simulink model "DataCenterCooling"  (R2026a)
settings: Solver=VariableStepAuto  StopTime=432000  AbsTol=1e-3
PreLoadFcn:
  | load DataCenterCoolingHeatLoad.mat
  | load DataCenterCoolingEnviornment.mat
  | 
  | % Chiller Setpoint
  | T_chiller = 18; % degC
  | 
  | % Pipes
  | server_pipe_D = 0.02; % m
  | server_pipe_L = 12; % m
  | server_pipe_thickness = 0.002; % m
  | server_num_pipes = 800;
  | 
  | % Material properties
  | rho_pipe = 7800; % kg/m^3
  | cp_pipe = 500; % J/(kg*K)
  | 
  | % Total connecting port areas
  | port_area = 0.2; % m^2
  | 
  | % Cooling tower
  | T_reservoir = 23; % degC
  | fan_area = 15; % m^2
  | tower_height = 3; % m
  | tower_area = 15; % m^2
libraries: fl_lib x38, nesl_utility x24, SimscapeFluids_lib x14, simulink_extras x2, slpidlib x2
(part 2 of 2)

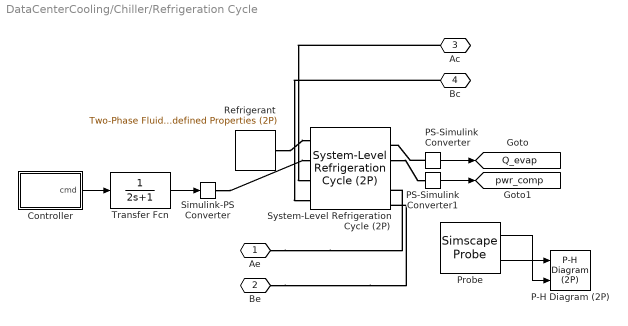
== system DataCenterCooling/Chiller/Refrigeration Cycle ==
  Controller : Subsystem
  P-H Diagram (2P) : SimscapeFluids_lib/Two-Phase Fluid/Utilities/P-H Diagram (2P)  p_unit=MPa  h_unit=kJ/kg
  PS-Simulink Converter : nesl_utility/PS-Simulink Converter  PhysicalDomain=network_engine_domain  SubClassName=ps_output  LeftPortType=input  RightPortType=output  PseudoPeriodic=off  Frequencies=[]  VectorFormat=inherit  Unit=kW  AffineConversion=off
  PS-Simulink Converter1 : nesl_utility/PS-Simulink Converter  PhysicalDomain=network_engine_domain  SubClassName=ps_output  LeftPortType=input  RightPortType=output  PseudoPeriodic=off  Frequencies=[]  VectorFormat=inherit  Unit=kW  AffineConversion=off
  Probe : SimscapeProbe  BoundBlock=48  Variables={h_cycle, p_cycle}
  Refrigerant : SimscapeFluids_lib/Two-Phase Fluid/Utilities/Two-Phase Fluid Predefined Properties (2P)  fluid=fluids.two_phase_fluid.utilities.enum.Fluid.R134a  p_atm=0.101325 MPa  properties_range_check=simscape.enum.assert.action.error  q_rev=0.01 Pa
  Simulink-PS Converter : nesl_utility/Simulink-PS Converter  PhysicalDomain=network_engine_domain  SubClassName=ps_input  LeftPortType=input  RightPortType=output  PseudoPeriodic=off  Frequencies=[]  NoiseDistribution=none  NoiseParameters=[]  Unit=1  AffineConversion=off  FilteringAndDerivatives=provide  SimscapeFilterOrder=1  InputFilterTimeConstant=0.001  UdotUserProvided=0
  System-Level Refrigeration Cycle (2P) : SimscapeFluids_lib/Two-Phase Fluid/Thermodynamic Cycles/System-Level Refrigeration Cycle (2P)  capacity_spec=fluids.two_phase_fluid.thermodynamic_cycles.enum.RefrigerationCycleCapacitySpec.CoolingLoad  Q_cond_nominal=15 kW  Q_evap_nominal=3500 kW  mdot_nominal=0.005 kg/s  pressure_spec=fluids.two_phase_fluid.thermodynamic_cycles.enum.RefrigerationCyclePressureSpec.SaturationTemperature  p_cond_nominal=1 MPa  p_evap_nominal=0.1 MPa  T_cond_nominal=30 degC  T_evap_nominal=16 degC  delta_T_sub_nominal=2 deltaK  delta_T_sup_nominal=5 deltaK  delta_T_sup_static=2 deltaK  performance_spec=fluids.two_phase_fluid.thermodynamic_cycles.enum.RefrigerationCyclePerformanceSpec.CompressorEfficiency  COP_nominal=3  comp_eta_s=0.8  comp_eta_v_nominal=0.9  comp_eta_m=0.95  valve_max_fraction=1.5  valve_leak_fraction=1e-6  valve_smoothing_factor=0.01  volume_cond=0.75 m^3  volume_evap=0.75 m^3  receiver_volume=1 m^3  receiver_L_init=0.4  nominal_init=true  p_cond_init=1 MPa  p_evap_init=0.1 MPa  h_cond_init=[450, 250] kJ/kg  h_evap_init=[250, 400] kJ/kg  receiver_saturated_init=true  receiver_h_liq_init=500 kJ/kg  receiver_h_vap_init=3500 kJ/kg  cond_domain=fluids.two_phase_fluid.thermodynamic_cycles.enum.RefrigerationCycleFluidDomain.ThermalLiquid  cond_mdot_nominal=250 kg/s  cond_delta_p_nominal=0.1 MPa  cond_pressure_spec=fluids.two_phase_fluid.thermodynamic_cycles.enum.RefrigerationCyclePressureSpec.Pressure  cond_p_in_nominal=0.2 MPa  cond_T_sat_nominal=400 K  cond_inlet_spec=fluids.two_phase_fluid.thermodynamic_cycles.enum.RefrigerationCycleInletSpec.Enthalpy  cond_T_in_nominal=26 degC  cond_h_in_nominal=500 kJ/kg  cond_x_in_nominal=1  cond_inlet_humidity_spec=foundation.enum.HumiditySpec.RelativeHumidity  cond_RH_in_nominal=0.1  cond_x_w_in_nominal=0.01  cond_y_w_in_nominal=0.01  cond_HR_in_nominal=0.01  cond_Tw_in_nominal=287 K  cond_inlet_trace_gas_spec=foundation.enum.trace_gas_spec.mass_fraction  cond_x_g_in_nominal=0.001  cond_y_g_in_nominal=0.001  cond_volume=0.75 m^3  area_Ac=port_area m^2  area_Bc=port_area m^2  cond_wall_thermal_mass=true  cond_mass_wall=pi*0.016*10 * 370 * 0.002 * rho_pipe kg  cond_cp_wall=cp_pipe J/(K*kg)  cond_nominal_init=false  cond_p_init=0.101325 + 0.01 MPa  cond_energy_spec=foundation.enum.energy_spec.enthalpy  cond_T_init=28 degC  cond_x_init=0.5  cond_alpha_init=0.5  cond_h_init=1500 kJ/kg  cond_u_init=1500 kJ/kg  cond_humidity_spec=foundation.enum.HumiditySpec.RelativeHumidity  cond_RH_init=0.5  cond_x_w_init=0.01  cond_y_w_init=0.01  cond_HR_init=0.01  cond_Tw_init=287 K  cond_trace_gas_spec=foundation.enum.trace_gas_spec.mass_fraction  cond_x_g_init=0.001  cond_y_g_init=0.001  cond_r_d_init=0  cond_T_wall_init=28 degC  cond_RH_ws=1  cond_time_constant_cond=1e-3 s  cond_time_constant_evap=1e-3 s  cond_fraction_entrained=1  evap_domain=fluids.two_phase_fluid.thermodynamic_cycles.enum.RefrigerationCycleFluidDomain.ThermalLiquid  evap_mdot_nominal=185 kg/s  evap_delta_p_nominal=0.1 MPa  evap_pressure_spec=fluids.two_phase_fluid.thermodynamic_cycles.enum.RefrigerationCyclePressureSpec.Pressure  evap_p_in_nominal=0.55 MPa  evap_T_sat_nominal=400 K  evap_inlet_spec=fluids.two_phase_fluid.thermodynamic_cycles.enum.RefrigerationCycleInletSpec.Enthalpy  evap_T_in_nominal=23 degC  evap_h_in_nominal=500 kJ/kg  evap_x_in_nominal=1  evap_inlet_humidity_spec=foundation.enum.HumiditySpec.RelativeHumidity  evap_RH_in_nominal=0.1  evap_x_w_in_nominal=0.01  evap_y_w_in_nominal=0.01  evap_HR_in_nominal=0.01  evap_Tw_in_nominal=287 K  evap_inlet_trace_gas_spec=foundation.enum.trace_gas_spec.mass_fraction  evap_x_g_in_nominal=0.001  evap_y_g_in_nominal=0.001  evap_volume=0.75 m^3  area_Ae=port_area m^2  area_Be=port_area m^2  evap_wall_thermal_mass=true  evap_mass_wall=pi*0.016*10 * 370 * 0.002 * rho_pipe kg  evap_cp_wall=cp_pipe J/(K*kg)  evap_nominal_init=false  evap_p_init=0.4 MPa  evap_energy_spec=foundation.enum.energy_spec.enthalpy  evap_T_init=18 degC  evap_x_init=0.5  evap_alpha_init=0.5  evap_h_init=1500 kJ/kg  evap_u_init=1500 kJ/kg  evap_humidity_spec=foundation.enum.HumiditySpec.RelativeHumidity  evap_RH_init=0.5  evap_x_w_init=0.01  evap_y_w_init=0.01  evap_HR_init=0.01  evap_Tw_init=287 K  evap_trace_gas_spec=foundation.enum.trace_gas_spec.mass_fraction  evap_x_g_init=0.001  evap_y_g_init=0.001  evap_r_d_init=0  evap_T_wall_init=18 degC  evap_RH_ws=1  evap_time_constant_cond=1e-3 s  evap_time_constant_evap=1e-3 s  evap_fraction_entrained=1  cond_coeff_modify=false  cond_a_liq_refrig=0.023  cond_a_mix_refrig=0.005  cond_a_vap_refrig=0.023  cond_b_refrig=0.8  cond_c_refrig=0.33  cond_a_liq_extfld=0.023  cond_a_mix_extfld=0.005  cond_a_vap_extfld=0.023  cond_a_extfld=0.023  cond_b_extfld=0.8  cond_c_extfld=0.33  evap_coeff_modify=false  evap_a_liq_refrig=0.023  evap_a_mix_refrig=0.005  evap_a_vap_refrig=0.023  evap_b_refrig=0.8  evap_c_refrig=0.33  evap_a_liq_extfld=0.023  evap_a_mix_extfld=0.005  evap_a_vap_extfld=0.023  evap_a_extfld=0.023  evap_b_extfld=0.8  evap_c_extfld=0.33
  Transfer Fcn : TransferFcn  Denominator=[2 1]
  Ae : PMIOPort  Side=Left
  Be : PMIOPort  Port=2  Side=Left
  Ac : PMIOPort  Port=3  Side=Right
  Bc : PMIOPort  Port=4  Side=Right
  tag scope: Q_evap=global, pwr_comp=global
  wires:
  Transfer Fcn/1 -> Simulink-PS Converter/1
  Controller/1(cmd) -> Transfer Fcn/1
  PS-Simulink Converter/1 -> [Q_evap]
  PS-Simulink Converter1/1 -> [pwr_comp]
  Probe/2 -> P-H Diagram (2P)/1
  Probe/1 -> P-H Diagram (2P)/2
  connections:
  Ae/RConn1 -- System-Level Refrigeration Cycle (2P)/RConn5
  Be/RConn1 -- System-Level Refrigeration Cycle (2P)/RConn6
  Ac/RConn1 -- System-Level Refrigeration Cycle (2P)/LConn3
  Bc/RConn1 -- System-Level Refrigeration Cycle (2P)/LConn4
  Refrigerant/RConn1 -- System-Level Refrigeration Cycle (2P)/LConn1
  Simulink-PS Converter/RConn1 -- System-Level Refrigeration Cycle (2P)/LConn2
  PS-Simulink Converter/LConn1 -- System-Level Refrigeration Cycle (2P)/RConn2
  System-Level Refrigeration Cycle (2P)/RConn3 -- PS-Simulink Converter1/LConn1

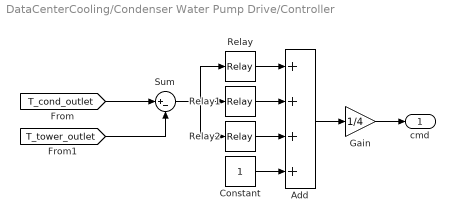
== system DataCenterCooling/Condenser Water Pump Drive/Controller ==
  Add : Sum  Inputs=++++
  Constant : Constant
  Gain : Gain  Gain=1/4
  Relay : Relay  OnSwitchValue=6  OffSwitchValue=4  ZeroCross=off
  Relay1 : Relay  OnSwitchValue=4  OffSwitchValue=2  ZeroCross=off
  Relay2 : Relay  OnSwitchValue=2  OffSwitchValue=0  ZeroCross=off
  Sum : Sum  Inputs=|+-
  cmd : Outport
  wires:
  Relay/1 -> Add/1
  Relay1/1 -> Add/2
  Relay2/1 -> Add/3
  Constant/1 -> Add/4
  Sum/1 -> Relay2/1, Relay1/1, Relay/1
  Add/1 -> Gain/1
  Gain/1 -> cmd/1
  [T_cond_outlet] -> Sum/1
  [T_tower_outlet] -> Sum/2

== system DataCenterCooling/Chiller/Abstract Model/Controller ==
  PID Controller : slpidlib/PID Controller  Controller=PI  Form=Parallel  TimeDomain=Continuous-time  UseExternalTs=off  SampleTime=-1  IntegratorMethod=Forward Euler  FilterMethod=Forward Euler  ControllerParametersSource=internal  P=0.1  I=0.01  UseKiTs=off  D=0  UseExternalDerivativeSource=off  N=100  UseFilter=on  TunerSelectOption=Transfer Function Based (PID Tuner App)  ZeroCross=off  InitialConditionSource=internal  InitialConditionForIntegrator=0  InitialConditionForFilter=0  DifferentiatorICPrevScaledInput=0  ExternalReset=none  TrackingMode=off  Kt=1  LimitOutput=off  SatLimitsSource=internal  UpperSaturationLimit=inf  LowerSaturationLimit=-inf  LinearizeAsGain=on  AntiWindupMode=none  Kb=1  LimitIntegrator=off  UpperIntegratorSaturationLimit=inf  LowerIntegratorSaturationLimit=-inf  POutMin=[]  POutMax=[]  IOutMin=[]  IOutMax=[]  DOutMin=[]  DOutMax=[]  NOutMin=[]  NOutMax=[]  SumOutMin=[]  SumOutMax=[]  SaturationOutMin=[]  SaturationOutMax=[]  PParamMin=[]  PParamMax=[]  IParamMin=[]  IParamMax=[]  DParamMin=[]  DParamMax=[]  NParamMin=[]  NParamMax=[]  KbParamMin=[]  KbParamMax=[]  KtParamMin=[]  KtParamMax=[]  KbOutMin=[]  KbOutMax=[]  KtOutMin=[]  KtOutMax=[]  IntegratorOutMin=[]  IntegratorOutMax=[]  FilterOutMin=[]  FilterOutMax=[]  SumI1OutMin=[]  SumI1OutMax=[]  SumI2OutMin=[]  SumI2OutMax=[]  SumI3OutMin=[]  SumI3OutMax=[]  SumI4OutMin=[]  SumI4OutMax=[]  SumDOutMin=[]  SumDOutMax=[]  DifferentiatorOutMin=[]  DifferentiatorOutMax=[]  FilterDiffOutCoefMin=[]  FilterDiffOutCoefMax=[]  ReciprocalOutMin=[]  ReciprocalOutMax=[]  SumDenOutMin=[]  SumDenOutMax=[]  SumNumOutMin=[]  SumNumOutMax=[]  DivideOutMin=[]  DivideOutMax=[]  UdiffTsProdOutMin=[]  UdiffTsProdOutMax=[]  NTsProdOutMin=[]  NTsProdOutMax=[]  UintegralTsProdOutMin=[]  UintegralTsProdOutMax=[]  UngainTsProdOutMin=[]  UngainTsProdOutMax=[]  ClampingZeroOutDataTypeStr=Inherit: Inherit via back propagation  ClampingZeroOutMin=[]  ClampingZeroOutMax=[]  FilterDenConstantOutDataTypeStr=Inherit: Inherit via back propagation  FilterDenConstantOutMin=[]  FilterDenConstantOutMax=[]  PCopyOutDataTypeStr=Inherit: Inherit via back propagation  PCopyOutMin=[]  PCopyOutMax=[]  NCopyOutDataTypeStr=Inherit: Inherit via back propagation  NCopyOutMin=[]  NCopyOutMax=[]  IntegratorContinuousStateAttributes=''  IntegratorStateMustResolveToSignalObject=off  IntegratorRTWStateStorageClass=Auto  FilterContinuousStateAttributes=''  FilterStateMustResolveToSignalObject=off  FilterRTWStateStorageClass=Auto  ParallelPVariant=InternalParameters  IdealPVariant=Disabled  IVariant=InternalParameters  DVariant=Disabled  IntegratorVariant=Continuous  SatVariant=Disabled  AWVariant=Passthrough  PCopyVariant=Disabled  TRVariant=Disabled  FdbkBlocksVariant=Forward  IdealPFdbkVariant=Disabled  SatFdbkVariant=Disabled  DerivativeFilterVariant=Disabled  NVariant=Disabled  NCopyVariant=Disabled_SignalSpec  FilterICVariant=Disabled  IntegratorICVariant=InternalICs  ExternalResetVariant=Disabled  TRSumVariant=Passthrough  SumFdbkVariant=Disabled  SumVariant=Sum_PI  TsampFilterVariant=InternalTs  TsampNgainVariant=Passthrough  TsampIntegralVariant=Disabled_SignalSpec  ExternalSaturationOutDataTypeStr=Inherit: Same as second input  DerivativeSourceVariant=Disabled  PreIntVariant=InternalPreInt
  Setpoint : Constant  Value=T_chiller
  Sum : Sum  Inputs=|+-
  cmd : Outport
  wires:
  PID Controller/1 -> cmd/1
  [T_evap_outlet] -> Sum/1
  Setpoint/1 -> Sum/2
  Sum/1 -> PID Controller/1

== system DataCenterCooling/Chiller/Refrigeration Cycle/Controller ==
  PID Controller : slpidlib/PID Controller  Controller=PI  Form=Parallel  TimeDomain=Continuous-time  UseExternalTs=off  SampleTime=-1  IntegratorMethod=Forward Euler  FilterMethod=Forward Euler  ControllerParametersSource=internal  P=0.1  I=0.01  UseKiTs=off  D=0  UseExternalDerivativeSource=off  N=100  UseFilter=on  TunerSelectOption=Transfer Function Based (PID Tuner App)  ZeroCross=off  InitialConditionSource=internal  InitialConditionForIntegrator=0  InitialConditionForFilter=0  DifferentiatorICPrevScaledInput=0  ExternalReset=none  TrackingMode=off  Kt=1  LimitOutput=off  SatLimitsSource=internal  UpperSaturationLimit=inf  LowerSaturationLimit=-inf  LinearizeAsGain=on  AntiWindupMode=none  Kb=1  LimitIntegrator=off  UpperIntegratorSaturationLimit=inf  LowerIntegratorSaturationLimit=-inf  POutMin=[]  POutMax=[]  IOutMin=[]  IOutMax=[]  DOutMin=[]  DOutMax=[]  NOutMin=[]  NOutMax=[]  SumOutMin=[]  SumOutMax=[]  SaturationOutMin=[]  SaturationOutMax=[]  PParamMin=[]  PParamMax=[]  IParamMin=[]  IParamMax=[]  DParamMin=[]  DParamMax=[]  NParamMin=[]  NParamMax=[]  KbParamMin=[]  KbParamMax=[]  KtParamMin=[]  KtParamMax=[]  KbOutMin=[]  KbOutMax=[]  KtOutMin=[]  KtOutMax=[]  IntegratorOutMin=[]  IntegratorOutMax=[]  FilterOutMin=[]  FilterOutMax=[]  SumI1OutMin=[]  SumI1OutMax=[]  SumI2OutMin=[]  SumI2OutMax=[]  SumI3OutMin=[]  SumI3OutMax=[]  SumI4OutMin=[]  SumI4OutMax=[]  SumDOutMin=[]  SumDOutMax=[]  DifferentiatorOutMin=[]  DifferentiatorOutMax=[]  FilterDiffOutCoefMin=[]  FilterDiffOutCoefMax=[]  ReciprocalOutMin=[]  ReciprocalOutMax=[]  SumDenOutMin=[]  SumDenOutMax=[]  SumNumOutMin=[]  SumNumOutMax=[]  DivideOutMin=[]  DivideOutMax=[]  UdiffTsProdOutMin=[]  UdiffTsProdOutMax=[]  NTsProdOutMin=[]  NTsProdOutMax=[]  UintegralTsProdOutMin=[]  UintegralTsProdOutMax=[]  UngainTsProdOutMin=[]  UngainTsProdOutMax=[]  ClampingZeroOutDataTypeStr=Inherit: Inherit via back propagation  ClampingZeroOutMin=[]  ClampingZeroOutMax=[]  FilterDenConstantOutDataTypeStr=Inherit: Inherit via back propagation  FilterDenConstantOutMin=[]  FilterDenConstantOutMax=[]  PCopyOutDataTypeStr=Inherit: Inherit via back propagation  PCopyOutMin=[]  PCopyOutMax=[]  NCopyOutDataTypeStr=Inherit: Inherit via back propagation  NCopyOutMin=[]  NCopyOutMax=[]  IntegratorContinuousStateAttributes=''  IntegratorStateMustResolveToSignalObject=off  IntegratorRTWStateStorageClass=Auto  FilterContinuousStateAttributes=''  FilterStateMustResolveToSignalObject=off  FilterRTWStateStorageClass=Auto  ParallelPVariant=InternalParameters  IdealPVariant=Disabled  IVariant=InternalParameters  DVariant=Disabled  IntegratorVariant=Continuous  SatVariant=Disabled  AWVariant=Passthrough  PCopyVariant=Disabled  TRVariant=Disabled  FdbkBlocksVariant=Forward  IdealPFdbkVariant=Disabled  SatFdbkVariant=Disabled  DerivativeFilterVariant=Disabled  NVariant=Disabled  NCopyVariant=Disabled_SignalSpec  FilterICVariant=Disabled  IntegratorICVariant=InternalICs  ExternalResetVariant=Disabled  TRSumVariant=Passthrough  SumFdbkVariant=Disabled  SumVariant=Sum_PI  TsampFilterVariant=InternalTs  TsampNgainVariant=Passthrough  TsampIntegralVariant=Disabled_SignalSpec  ExternalSaturationOutDataTypeStr=Inherit: Same as second input  DerivativeSourceVariant=Disabled  PreIntVariant=InternalPreInt
  Setpoint : Constant  Value=T_chiller
  Sum : Sum  Inputs=|+-
  cmd : Outport
  wires:
  PID Controller/1 -> cmd/1
  [T_evap_outlet] -> Sum/1
  Setpoint/1 -> Sum/2
  Sum/1 -> PID Controller/1
